simulink model "YMBOX_Deluxe_sim"  (R2024b)
settings: Solver=FixedStepDiscrete  StartTime=0.0  StopTime=YMBOX_Drive_Config.Execution.StopTime_s  FixedStep=KfSIM_PowerStageStep_s  RelTol=1e-3
PreLoadFcn:
  | run(fullfile(fileparts(get_param(bdroot,'FileName')), 'YMBOX_Deluxe_init.m'));
InitFcn:
  | YMBOX_InitializeModel('simulation',bdroot);
model workspace (MAT data in the model file):
  KfMDSP_DCBusVoltFilterCutoff_Hz = Simulink.Parameter
  KfMDSP_DCBusVoltFilterCutoff_Hz.Value = 500
  KfMDSP_DCBusVoltFilterCutoff_Hz.Complexity = 'real'
  KfMDSP_DCBusVoltFilterCutoff_Hz.Dimensions = [1 1]
  KfMDSP_DCBusVoltFilterCutoff_Hz.Description = 'DC bus voltage low-pass cutoff frequency in Hz'
  KfMDSP_DCBusVoltFilterCutoff_Hz.DataType = 'single'
  KfMDSP_DCBusVoltFilterCutoff_Hz.Min = 10
  KfMDSP_DCBusVoltFilterCutoff_Hz.Max = 1000
undefined symbols (not defined in the file or in its folder): Cf_CONTROL_TASK_TIME_S, Cf_TICK_TIME_S, KfPLL_PositionCountsPerRev_NULL, KfSIM_PowerStageStep_s, KfSIM_PwmPeriod_s, KuSIM_PwmDeadTimeSteps_NULL, YMBOX_Drive_Config
libraries: simulink x3, spsDCVoltageSourceLib x1, spsPermanentMagnetSynchronousMachineLib x1, spsUniversalBridgeLib x1, spspowerguiLib x1
CloseFcn:
  | YMBOX_Deluxe_exit
settings Model: Creator=ASUS  LastModifiedBy=ASUS
settings SolverCC: AlgebraicLoopSolver=TrustRegion  AutoInsertRateTranBlk=on
settings DataIOCC: LimitDataPoints=on  SaveFormat=StructureWithTime  SignalLoggingSaveFormat=ModelDataLogs  SaveOutput=off  SaveTime=off  ReturnWorkspaceOutputs=off
settings OptimizationCC: BlockReduction=off  ConditionallyExecuteInputs=off  DefaultParameterBehavior=Inlined  EnhancedBackFolding=on  PassReuseOutputArgsAs=Individual arguments  ExpressionDepthLimit=2147483647  ZeroExternalMemoryAtStartup=off  ZeroInternalMemoryAtStartup=off  InitFltsAndDblsToZero=on  EfficientFloat2IntCast=on  EfficientMapNaN2IntZero=off  OptimizeBlockOrder=speed  DifferentSizesBufferReuse=on  OptimizationCustomize=off  EfficientTunableParamExpr=on
settings DebuggingCC: ConsistencyChecking=warning  ArrayBoundsChecking=error  SignalInfNanChecking=error  SignalRangeChecking=error  SaveWithParameterizedLinksMsg=none  CheckSSInitialOutputMsg=off  UnderspecifiedInitializationDetection=Classic  MergeDetectMultiDrivingBlocksExec=none  TimeAdjustmentMsg=warning  MaxConsecutiveZCsMsg=warning  SolverPrmCheckMsg=warning  InheritedTsInSrcMsg=none  CheckMatrixSingularityMsg=error  ParameterOverflowMsg=warning  ParameterUnderflowMsg=error  ParameterPrecisionLossMsg=none  ParameterTunabilityLossMsg=error  FixptConstUnderflowMsg=warning  FixptConstOverflowMsg=warning  FixptConstPrecisionLossMsg=warning  VectorMatrixConversionMsg=warning  FcnCallInpInsideContextMsg=warning  UnconnectedInputMsg=warning  UnconnectedOutputMsg=warning  UnconnectedLineMsg=warning  UniqueDataStoreMsg=warning  AllowSymbolicDim=off  StateNameClashWarn=warning  SFUnexpectedBacktrackingDiag=warning  SFNoUnconditionalDefaultTransitionDiag=warning  SFExecutionAtInitializationDiag=none  ArithmeticOperatorsInVariantConditions=warning
settings HardwareCC: ProdBitPerPointer=32  ProdBitPerSizeT=32  ProdBitPerPtrDiffT=32  ProdLargestAtomicFloat=None  ProdWordSize=32  ProdHWDeviceType=Infineon->TriCore  TargetIntDivRoundTo=Zero  TargetEndianess=LittleEndian  TargetHWDeviceType=Infineon->TriCore  ProdEqTarget=off
settings ModelReferenceCC: EnableRefExpFcnMdlSchedulingChecks=on  PropagateSignalLabelsOutOfModel=off
settings SFSimCC: SimUseLocalCustomCode=off  MATLABDynamicMemAlloc=off  CustomCodeUndefinedFunction=UseInterfaceOnly
settings SFSimCC: SimCustomSourceCode=|
  | void Pwm_SetOutputToIdle_Now(void){};
  | void InverterDisable(void){};
  | void Pwm_Write(void){};
  | void InverterEnable(void){};
  | void vPwm_MDCC_UdUqCalc1_PI_Self_initialize(void){};
  | void SpeedLoopMode_initialize(void){};
settings SFSimCC: SimCustomHeaderCode=|
  | void Pwm_SetOutputToIdle_Now(void);
  | void InverterDisable(void);
  | void Pwm_Write(void);
  | void InverterEnable(void);
  | void vPwm_MDCC_UdUqCalc1_PI_Self_initialize(void);
  | void SpeedLoopMode_initialize(void);
settings RTWCC: Description=Embedded Coder  SystemTargetFile=ert.tlc  TLCOptions=-p0  GenCodeOnly=on  TemplateMakefile=ert_default_tmf  GenerateReport=on  RTWUseLocalCustomCode=off  IncludeHyperlinkInReport=on  LaunchReport=on  GPUComputeCapability=3.5
settings RTWCC: CustomHeaderCode=|
  | extern void Pwm_SetOutputToIdle_Now(void);
  | extern void InverterDisable(void);
  | extern void Pwm_Write(void);
  | extern void InverterEnable(void);
  | void vPwm_MDCC_UdUqCalc1_PI_Self_initialize(void);
  | void SpeedLoopMode_initialize(void);
settings CodeAppCC: ForceParamTrailComments=on  IgnoreCustomStorageClasses=off  MaxIdLength=100  OperatorAnnotations=on  SimulinkDataObjDesc=on  SFDataObjDesc=on  CustomSymbolStrGlobalVar=rt$N$M  CustomSymbolStrType=$N$M  CustomSymbolStrFcn=$N$M$F  CustomSymbolStrMacro=$N$M  CustomCommentsFcn=comments_mptfun.m  DefineNamingRule=UpperCase  InsertBlockDesc=on  InternalIdentifier=Classic
settings ERTTargetCC: GenerateSampleERTMain=on  ERTCustomFileTemplate=example_file_process.tlc
settings ConfigComp: CovMetricSettings=dw  CovSaveCumulativeToWorkspaceVar=on  CovSaveSingleToWorkspaceVar=on  CovExternalEMLEnable=off

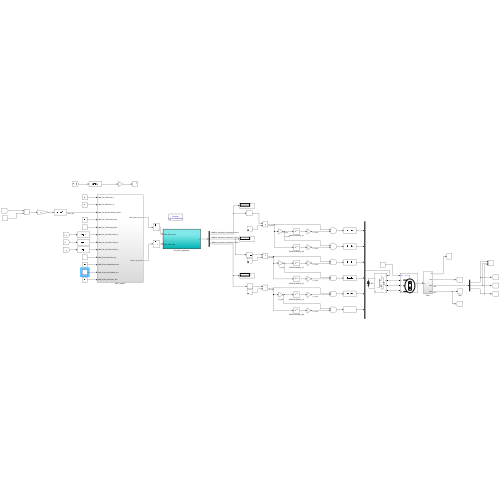
[thumbnail: Simulink's stored preview of the top-level diagram]
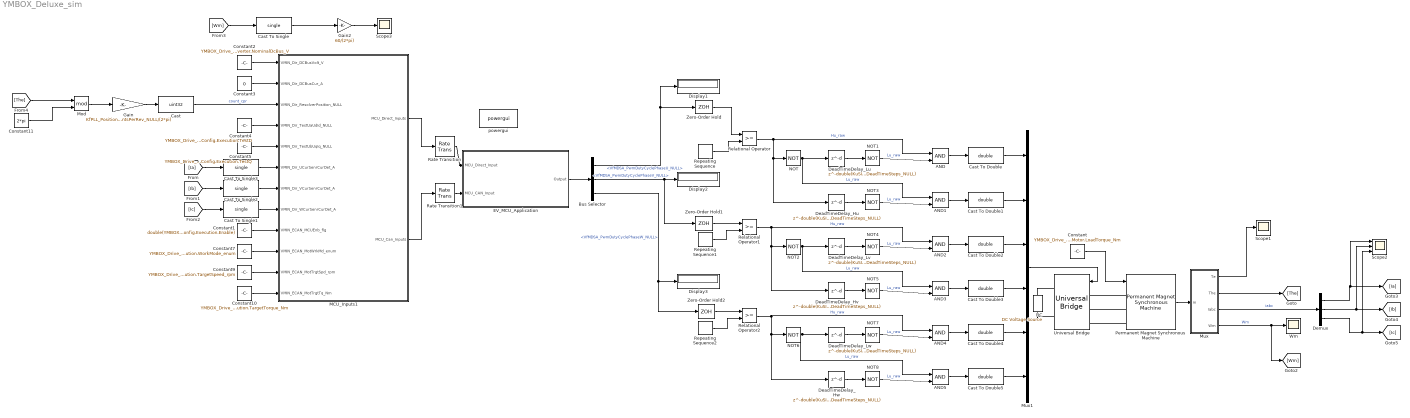
== system YMBOX_Deluxe_sim ==
  AND{,1..5} (6 alike) : Logic  IconShape=distinctive  AllPortsSameDT=off  OutDataTypeStr=boolean
  Bus Selector : BusSelector  OutputSignals=MDSA_output.VfMDSA_PwmDutyCyclePhaseU_NULL,MDSA_output.VfMDSA_PwmDutyCyclePhaseV_NULL,MDSA_output.VfMDSA_PwmDutyCyclePhaseW_NULL
  Cast : DataTypeConversion  OutDataTypeStr=uint32  SaturateOnIntegerOverflow=off  RndMeth=Floor
  Cast To Double{,1..5} (6 alike) : DataTypeConversion  OutDataTypeStr=double  SaturateOnIntegerOverflow=off  RndMeth=Floor
  Cast To Single{,1..3} (4 alike) : DataTypeConversion  OutDataTypeStr=single  SaturateOnIntegerOverflow=off  RndMeth=Floor
  Constant : Constant  Value=YMBOX_Drive_Config.Motor.LoadTorque_Nm
  Constant1 : Constant  Value=double(YMBOX_Drive_Config.Execution.Enable)  OutDataTypeStr=boolean
  Constant10 : Constant  Value=YMBOX_Drive_Config.Execution.TargetTorque_Nm  OutDataTypeStr=single
  Constant11 : Constant  Value=2*pi
  Constant2 : Constant  Value=YMBOX_Drive_Config.Inverter.NominalDcBus_V  OutDataTypeStr=single
  Constant3 : Constant  Value=0  OutDataTypeStr=single
  Constant4 : Constant  Value=YMBOX_Drive_Config.Execution.TestD  OutDataTypeStr=single
  Constant5 : Constant  Value=YMBOX_Drive_Config.Execution.TestQ  OutDataTypeStr=single
  Constant7 : Constant  Value=YMBOX_Drive_Config.Execution.WorkMode_enum  OutDataTypeStr=uint16
  Constant9 : Constant  Value=YMBOX_Drive_Config.Execution.TargetSpeed_rpm  OutDataTypeStr=single
  DC : spsDCVoltageSourceLib/DC Voltage Source  Amplitude=YMBOX_Drive_Config.Inverter.NominalDcBus_V  Measurements=None
  DeadTimeDelay_Hu : Delay  DelayLength=double(KuSIM_PwmDeadTimeSteps_NULL)  InitialCondition=0  SampleTime=KfSIM_PowerStageStep_s
  DeadTimeDelay_Hv : Delay  DelayLength=double(KuSIM_PwmDeadTimeSteps_NULL)  InitialCondition=0  SampleTime=KfSIM_PowerStageStep_s
  DeadTimeDelay_Hw : Delay  DelayLength=double(KuSIM_PwmDeadTimeSteps_NULL)  InitialCondition=0  SampleTime=KfSIM_PowerStageStep_s
  DeadTimeDelay_Lu : Delay  DelayLength=double(KuSIM_PwmDeadTimeSteps_NULL)  InitialCondition=0  SampleTime=KfSIM_PowerStageStep_s
  DeadTimeDelay_Lv : Delay  DelayLength=double(KuSIM_PwmDeadTimeSteps_NULL)  InitialCondition=0  SampleTime=KfSIM_PowerStageStep_s
  DeadTimeDelay_Lw : Delay  DelayLength=double(KuSIM_PwmDeadTimeSteps_NULL)  InitialCondition=0  SampleTime=KfSIM_PowerStageStep_s
  Demux : Demux  Outputs=3
  Display1 : Display
  Display2 : Display
  Display3 : Display
  EV_MCU_Application : Subsystem  TreatAsAtomicUnit=on
      settings: RTWSystemCode=Nonreusable function  RTWFcnNameOpts=Use subsystem name  RTWFileNameOpts=Use subsystem name
  Gain : Gain  Gain=KfPLL_PositionCountsPerRev_NULL/(2*pi)
  Gain2 : Gain  Gain=60/(2*pi)
  MCU_Inputs1 : Subsystem
      settings: RTWSystemCode=Nonreusable function  RTWFcnNameOpts=Use subsystem name  RTWFileNameOpts=Use subsystem name
  Mod : Math  Operator=mod
  Mux : Subsystem
  Mux1 : Mux  Inputs=6
  NOT{,1..8} (9 alike) : Logic  Operator=NOT  IconShape=distinctive  AllPortsSameDT=off  OutDataTypeStr=boolean
  Permanent Magnet Synchronous Machine : spsPermanentMagnetSynchronousMachineLib/Permanent Magnet Synchronous Machine  NbPhases=3  FluxDistribution=Sinusoidal  RotorType=Salient-pole  MechanicalLoad=Torque Tm  PresetModel=No  ShowDetailedParameters=on  MeasurementBus=off  Resistance=YMBOX_Drive_Config.Motor.StatorResistance_Ohm  Inductance=8.5e-3  dqInductances=[YMBOX_Drive_Config.Motor.Ld_H YMBOX_Drive_Config.Motor.Lq_H]  La=YMBOX_Drive_Config.Motor.Ld_H  MachineConstant=Flux linkage established by magnets (V.s)  Flux=YMBOX_Drive_Config.Motor.PmFlux_Wb  VoltageCst=68.3065  TorqueCst=0.56489  Flat=120  Mechanical=[YMBOX_Drive_Config.Motor.Inertia_kgm2 YMBOX_Drive_Config.Motor.ViscousFriction_Nms YMBOX_Drive_Config.Motor.PolePairs 0]  PolePairs=YMBOX_Drive_Config.Motor.PolePairs  InitialConditions=[0,0, 0,0]  InitialConditions5ph=[0 0 0 0 0 0]  RefAngle=Aligned with phase A axis (original Park)  IterativeDiscreteModel=Trapezoidal non iterative  TsBlock=-1  TsPowergui=0
  Rate Transition : RateTransition  OutPortSampleTime=Cf_CONTROL_TASK_TIME_S
  Rate Transition1 : RateTransition  OutPortSampleTime=Cf_CONTROL_TASK_TIME_S
  Relational Operator : RelationalOperator  OutDataTypeStr=boolean  RndMeth=Simplest  InputSameDT=off
  Relational Operator1 : RelationalOperator  OutDataTypeStr=boolean  RndMeth=Simplest  InputSameDT=off
  Relational Operator2 : RelationalOperator  OutDataTypeStr=boolean  RndMeth=Simplest  InputSameDT=off
  Repeating Sequence : simulink/Sources/Repeating Sequence  rep_seq_t=[0 0.5*KfSIM_PwmPeriod_s KfSIM_PwmPeriod_s]  rep_seq_y=[0 1 0]
  Repeating Sequence1 : simulink/Sources/Repeating Sequence  rep_seq_t=[0 0.5*KfSIM_PwmPeriod_s KfSIM_PwmPeriod_s]  rep_seq_y=[0 1 0]
  Repeating Sequence2 : simulink/Sources/Repeating Sequence  rep_seq_t=[0 0.5*KfSIM_PwmPeriod_s KfSIM_PwmPeriod_s]  rep_seq_y=[0 1 0]
  Scope1 : Scope
  Scope2 : Scope  NumInputPorts=3
  Scope3 : Scope
  Universal Bridge : spsUniversalBridgeLib/Universal Bridge  Arms=3  SnubberResistance=1e5  SnubberCapacitance=inf  Device=IGBT / Diodes  Ron=1e-3  Lon=0  ForwardVoltages="[  0  0  ]"  ForwardVoltage=0  GTOparameters=[ 10e-6 , 20e-6 ]  IGBTparameters=[ 1e-6 , 2e-6 ]  Measurements=None  Measurements_2=None  converterType=Rectifier
  Wm : Scope
  Zero-Order Hold : ZeroOrderHold  SampleTime=Cf_CONTROL_TASK_TIME_S
  Zero-Order Hold1 : ZeroOrderHold  SampleTime=Cf_CONTROL_TASK_TIME_S
  Zero-Order Hold2 : ZeroOrderHold  SampleTime=Cf_CONTROL_TASK_TIME_S
  powergui : spspowerguiLib/powergui  Priority=1  SimulationMode=Discrete  SampleTime=KfSIM_PowerStageStep_s  frequency=60  Iterations=50  frequencyindice=0  Pbase=100e6  ErrMax=1e-4  UnitsV=kV  UnitsW=MW  buscounter=0  FunctionMessages=off  echomessages=off  EnableUseOfTLC=off  CurrentSourceSwitches=off  DisableSnubberDevices=off  DisableRonSwitches=off  DisableVfSwitches=off  DisplayEquations=off  AutomaticDiscreteSolvers=off  SolverType=Tustin/Backward Euler (TBE)  Interpol=off  ExternalGateDelay=off  methode=off  Ts=100  x0status=blocks  SPID=on  SwTol=0  HookPort=off  NonlinearTolerance=1e-4  nMaxIteration=100  ContinueOnMaxIteration=off  RestoreLinks=warning  ResistiveCurrentMeasurement=off  Frange=[0:2:500]  Ylog=off  Xlog=on  ShowGrid=off  save=off  variable=ZData  structure=0  ZoomFFT=off  StartTime=0.0  cycles=1  DisplayStyle=1  fundamental=60  FreqAxis=off  MaxFrequency=1000  frequencyindicesteady=1  RmsSteady=1  display=off
  wires:
  NOT6/1 -> AND5/1, DeadTimeDelay_Lw/1  "Lu_raw"
  Bus Selector/1 -> Display1/1, Zero-Order Hold/1  "<VfMDSA_PwmDutyCyclePhaseU_NULL>"
  Mux/4(Wm) -> [Wm], Wm/1  "Wm"
  [Ic] -> Cast To Single1/1
  Zero-Order Hold/1 -> Relational Operator/1
  Repeating Sequence2/1 -> Relational Operator2/2
  AND1/1 -> Cast To Double1/1
  AND/1 -> Cast To Double/1
  Mux/2(The) -> [The]
  [The] -> Mod/1
  Cast To Single/1 -> Gain2/1
  AND2/1 -> Cast To Double2/1
  Relational Operator1/1 -> AND2/1, DeadTimeDelay_Hv/1, NOT2/1  "Hu_raw"
  Demux/1 -> Scope2/1, [Ia]
  Relational Operator2/1 -> AND4/1, DeadTimeDelay_Hw/1, NOT6/1  "Hu_raw"
  Bus Selector/2 -> Zero-Order Hold1/1, Display2/1  "<VfMDSA_PwmDutyCyclePhaseV_NULL>"
  NOT8/1 -> AND5/2  "Lu_raw"
  NOT7/1 -> AND4/2  "Lu_raw"
  Cast To Double2/1 -> Mux1/3
  Cast To Single1/1 -> MCU_Inputs1/8(VMIN_Dir_WCurSenrCurDet_A)
  Constant3/1 -> MCU_Inputs1/2(VMIN_Dir_DCBusCur_A)
  Constant1/1 -> MCU_Inputs1/9(VMIN_ECAN_MCUEnb_flg)
  Zero-Order Hold1/1 -> Relational Operator1/1
  Constant/1 -> Permanent Magnet Synchronous Machine/1
  [Ib] -> Cast To Single2/1
  Constant5/1 -> MCU_Inputs1/5(VMIN_Dir_TestUbUqIq_NULL)
  NOT2/1 -> AND3/1, DeadTimeDelay_Lv/1  "Lu_raw"
  Gain2/1 -> Scope3/1
  Cast To Double/1 -> Mux1/1
  Constant10/1 -> MCU_Inputs1/12(VMIN_ECAN_MotTrgtTq_Nm)
  Cast To Single2/1 -> MCU_Inputs1/7(VMIN_Dir_VCurSenrCurDet_A)
  Permanent Magnet Synchronous Machine/1 -> Mux/1(m)
  Constant7/1 -> MCU_Inputs1/10(VMIN_ECAN_MotWrkMd_enum)
  Cast To Double1/1 -> Mux1/2
  Zero-Order Hold2/1 -> Relational Operator2/1
  Constant4/1 -> MCU_Inputs1/4(VMIN_Dir_TestUaUdId_NULL)
  Mux/1(Te) -> Scope1/1
  Demux/3 -> Scope2/3, [Ic]
  Constant2/1 -> MCU_Inputs1/1(VMIN_Dir_DCBusVolt_V)
  AND4/1 -> Cast To Double4/1
  Mod/1 -> Gain/1
  Cast To Double3/1 -> Mux1/4
  EV_MCU_Application/1(Output) -> Bus Selector/1
  NOT3/1 -> AND1/2  "Lu_raw"
  Demux/2 -> Scope2/2, [Ib]
  Cast To Single3/1 -> MCU_Inputs1/6(VMIN_Dir_UCurSenrCurDet_A)
  AND5/1 -> Cast To Double5/1
  NOT1/1 -> AND/2  "Lu_raw"
  Mux/3(Iabc) -> Demux/1  "iabc"
  Cast/1 -> MCU_Inputs1/3(VMIN_Dir_ResolverPosition_NULL)  "count_cpr"
  Gain/1 -> Cast/1
  Cast To Double5/1 -> Mux1/6
  NOT/1 -> AND1/1, DeadTimeDelay_Lu/1  "Lu_raw"
  Constant9/1 -> MCU_Inputs1/11(VMIN_ECAN_MotTrgtSpd_rpm)
  Mux1/1 -> Universal Bridge/1
  Constant11/1 -> Mod/2
  NOT4/1 -> AND2/2  "Lu_raw"
  Cast To Double4/1 -> Mux1/5
  NOT5/1 -> AND3/2  "Lu_raw"
  [Wm] -> Cast To Single/1
  Relational Operator/1 -> AND/1, DeadTimeDelay_Hu/1, NOT/1  "Hu_raw"
  Bus Selector/3 -> Zero-Order Hold2/1, Display3/1  "<VfMDSA_PwmDutyCyclePhaseW_NULL>"
  Repeating Sequence/1 -> Relational Operator/2
  AND3/1 -> Cast To Double3/1
  [Ia] -> Cast To Single3/1
  Repeating Sequence1/1 -> Relational Operator1/2
  MCU_Inputs1/1(MCU_Direct_Inputs) -> Rate Transition/1
  Rate Transition/1 -> EV_MCU_Application/1(MCU_Direct_Input)
  Rate Transition1/1 -> EV_MCU_Application/2(MCU_CAN_Input)
  MCU_Inputs1/2(MCU_Can_Inputs) -> Rate Transition1/1
  DeadTimeDelay_Lu/1 -> NOT1/1
  DeadTimeDelay_Hu/1 -> NOT3/1
  DeadTimeDelay_Lv/1 -> NOT4/1
  DeadTimeDelay_Hv/1 -> NOT5/1
  DeadTimeDelay_Lw/1 -> NOT7/1
  DeadTimeDelay_Hw/1 -> NOT8/1
  connections:
  DC/LConn1 -- Universal Bridge/RConn2
  DC/RConn1 -- Universal Bridge/RConn1
  Permanent Magnet Synchronous Machine/LConn3 -- Universal Bridge/LConn3
  Permanent Magnet Synchronous Machine/LConn1 -- Universal Bridge/LConn1
  Permanent Magnet Synchronous Machine/LConn2 -- Universal Bridge/LConn2

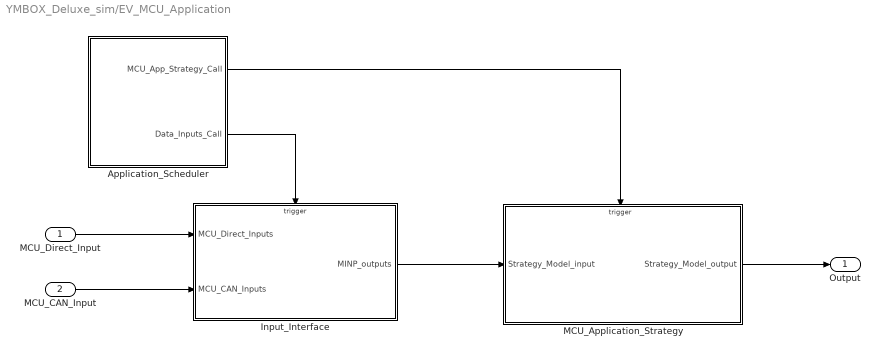
== system YMBOX_Deluxe_sim/EV_MCU_Application ==
  MCU_Direct_Input : Inport
  MCU_CAN_Input : Inport  Port=2
  Application_Scheduler : Subsystem
  Input_Interface : Subsystem
      settings: RTWSystemCode=Nonreusable function  RTWFcnNameOpts=Use subsystem name  RTWFileNameOpts=Use subsystem name
  MCU_Application_Strategy : Subsystem
      settings: RTWSystemCode=Nonreusable function  RTWFcnNameOpts=Use subsystem name  RTWFileNameOpts=Use subsystem name
  Output : Outport
  wires:
  MCU_Direct_Input/1 -> Input_Interface/1(MCU_Direct_Inputs)
  MCU_CAN_Input/1 -> Input_Interface/2(MCU_CAN_Inputs)
  Input_Interface/1(MINP_outputs) -> MCU_Application_Strategy/1(Strategy_Model_input)
  MCU_Application_Strategy/1(Strategy_Model_output) -> Output/1
  Application_Scheduler/1(MCU_App_Strategy_Call) -> MCU_Application_Strategy/Trigger
  Application_Scheduler/2(Data_Inputs_Call) -> Input_Interface/Trigger

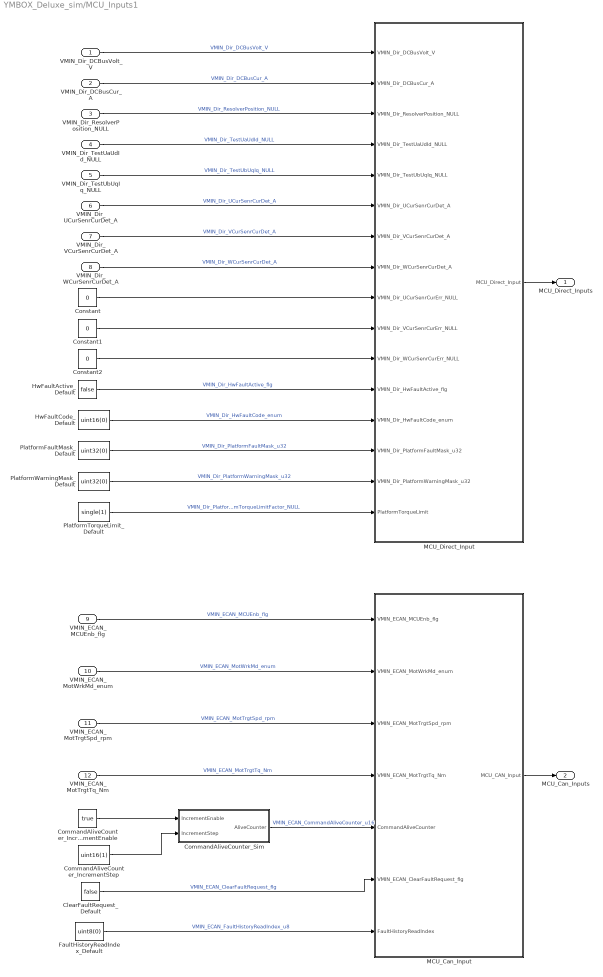
== system YMBOX_Deluxe_sim/MCU_Inputs1 ==
  VMIN_Dir_DCBusVolt_V : Inport
  VMIN_Dir_DCBusCur_A : Inport  Port=2
  VMIN_Dir_ResolverPosition_NULL : Inport  Port=3
  VMIN_Dir_TestUaUdId_NULL : Inport  Port=4
  VMIN_Dir_TestUbUqIq_NULL : Inport  Port=5
  VMIN_Dir_UCurSenrCurDet_A : Inport  Port=6
  VMIN_Dir_VCurSenrCurDet_A : Inport  Port=7
  VMIN_Dir_WCurSenrCurDet_A : Inport  Port=8
  VMIN_ECAN_MCUEnb_flg : Inport  Port=9
  VMIN_ECAN_MotWrkMd_enum : Inport  Port=10
  VMIN_ECAN_MotTrgtSpd_rpm : Inport  Port=11
  VMIN_ECAN_MotTrgtTq_Nm : Inport  Port=12
  ClearFaultRequest_Default : Constant  Value=false  OutDataTypeStr=boolean
  CommandAliveCounter_IncrementEnable : Constant  Description=仿真控制：true 时 AliveCounter 按步长递增；false 时保持当前值，用于触发 CommWatchdog 停更场景。  Value=true  OutDataTypeStr=boolean
  CommandAliveCounter_IncrementStep : Constant  Description=仿真控制：AliveCounter 每个控制节拍的 uint16 增量，默认 uint16(1)。  Value=uint16(1)  OutDataTypeStr=uint16
  CommandAliveCounter_Sim : Subsystem  Description=仿真专用命令存活计数器：Enable 有效时每个 Cf_TICK_TIME_S 加 IncrementStep；无效时保持；uint16 溢出自然回绕。
  Constant : Constant  Value=0  OutDataTypeStr=boolean
  Constant1 : Constant  Value=0  OutDataTypeStr=boolean
  Constant2 : Constant  Value=0  OutDataTypeStr=boolean
  FaultHistoryReadIndex_Default : Constant  Value=uint8(0)  OutDataTypeStr=uint8
  HwFaultActive_Default : Constant  Value=false  OutDataTypeStr=boolean
  HwFaultCode_Default : Constant  Value=uint16(0)  OutDataTypeStr=uint16
  MCU_Can_Input : Subsystem  TreatAsAtomicUnit=on
      settings: RTWSystemCode=Nonreusable function  RTWFcnNameOpts=Use subsystem name
  MCU_Direct_Input : Subsystem  TreatAsAtomicUnit=on
      settings: RTWSystemCode=Nonreusable function  RTWFcnNameOpts=Use subsystem name
  PlatformFaultMask_Default : Constant  Value=uint32(0)  OutDataTypeStr=uint32
  PlatformTorqueLimit_Default : Constant  Value=single(1)  OutDataTypeStr=single
  PlatformWarningMask_Default : Constant  Value=uint32(0)  OutDataTypeStr=uint32
  MCU_Direct_Inputs : Outport
  MCU_Can_Inputs : Outport  Port=2
  wires:
  VMIN_Dir_DCBusVolt_V/1 -> MCU_Direct_Input/1(VMIN_Dir_DCBusVolt_V)  "VMIN_Dir_DCBusVolt_V"
  VMIN_Dir_TestUbUqIq_NULL/1 -> MCU_Direct_Input/5(VMIN_Dir_TestUbUqIq_NULL)  "VMIN_Dir_TestUbUqIq_NULL"
  VMIN_Dir_TestUaUdId_NULL/1 -> MCU_Direct_Input/4(VMIN_Dir_TestUaUdId_NULL)  "VMIN_Dir_TestUaUdId_NULL"
  VMIN_Dir_ResolverPosition_NULL/1 -> MCU_Direct_Input/3(VMIN_Dir_ResolverPosition_NULL)  "VMIN_Dir_ResolverPosition_NULL"
  VMIN_Dir_DCBusCur_A/1 -> MCU_Direct_Input/2(VMIN_Dir_DCBusCur_A)  "VMIN_Dir_DCBusCur_A"
  VMIN_ECAN_MotTrgtTq_Nm/1 -> MCU_Can_Input/4(VMIN_ECAN_MotTrgtTq_Nm)  "VMIN_ECAN_MotTrgtTq_Nm"
  HwFaultCode_Default/1 -> MCU_Direct_Input/13(VMIN_Dir_HwFaultCode_enum)  "VMIN_Dir_HwFaultCode_enum"
  Constant1/1 -> MCU_Direct_Input/10(VMIN_Dir_VCurSenrCurErr_NULL)
  VMIN_Dir_WCurSenrCurDet_A/1 -> MCU_Direct_Input/8(VMIN_Dir_WCurSenrCurDet_A)  "VMIN_Dir_WCurSenrCurDet_A"
  HwFaultActive_Default/1 -> MCU_Direct_Input/12(VMIN_Dir_HwFaultActive_flg)  "VMIN_Dir_HwFaultActive_flg"
  Constant/1 -> MCU_Direct_Input/9(VMIN_Dir_UCurSenrCurErr_NULL)
  VMIN_Dir_VCurSenrCurDet_A/1 -> MCU_Direct_Input/7(VMIN_Dir_VCurSenrCurDet_A)  "VMIN_Dir_VCurSenrCurDet_A"
  VMIN_Dir_UCurSenrCurDet_A/1 -> MCU_Direct_Input/6(VMIN_Dir_UCurSenrCurDet_A)  "VMIN_Dir_UCurSenrCurDet_A"
  MCU_Can_Input/1(MCU_CAN_Input) -> MCU_Can_Inputs/1
  VMIN_ECAN_MCUEnb_flg/1 -> MCU_Can_Input/1(VMIN_ECAN_MCUEnb_flg)  "VMIN_ECAN_MCUEnb_flg"
  Constant2/1 -> MCU_Direct_Input/11(VMIN_Dir_WCurSenrCurErr_NULL)
  PlatformFaultMask_Default/1 -> MCU_Direct_Input/14(VMIN_Dir_PlatformFaultMask_u32)  "VMIN_Dir_PlatformFaultMask_u32"
  PlatformWarningMask_Default/1 -> MCU_Direct_Input/15(VMIN_Dir_PlatformWarningMask_u32)  "VMIN_Dir_PlatformWarningMask_u32"
  PlatformTorqueLimit_Default/1 -> MCU_Direct_Input/16(PlatformTorqueLimit)  "VMIN_Dir_PlatformTorqueLimitFactor_NULL"
  FaultHistoryReadIndex_Default/1 -> MCU_Can_Input/7(FaultHistoryReadIndex)  "VMIN_ECAN_FaultHistoryReadIndex_u8"
  VMIN_ECAN_MotWrkMd_enum/1 -> MCU_Can_Input/2(VMIN_ECAN_MotWrkMd_enum)  "VMIN_ECAN_MotWrkMd_enum"
  VMIN_ECAN_MotTrgtSpd_rpm/1 -> MCU_Can_Input/3(VMIN_ECAN_MotTrgtSpd_rpm)  "VMIN_ECAN_MotTrgtSpd_rpm"
  ClearFaultRequest_Default/1 -> MCU_Can_Input/6(VMIN_ECAN_ClearFaultRequest_flg)  "VMIN_ECAN_ClearFaultRequest_flg"
  MCU_Direct_Input/1(MCU_Direct_Input) -> MCU_Direct_Inputs/1
  CommandAliveCounter_IncrementEnable/1 -> CommandAliveCounter_Sim/1(IncrementEnable)
  CommandAliveCounter_IncrementStep/1 -> CommandAliveCounter_Sim/2(IncrementStep)
  CommandAliveCounter_Sim/1(AliveCounter) -> MCU_Can_Input/5(CommandAliveCounter)  "VMIN_ECAN_CommandAliveCounter_u16"

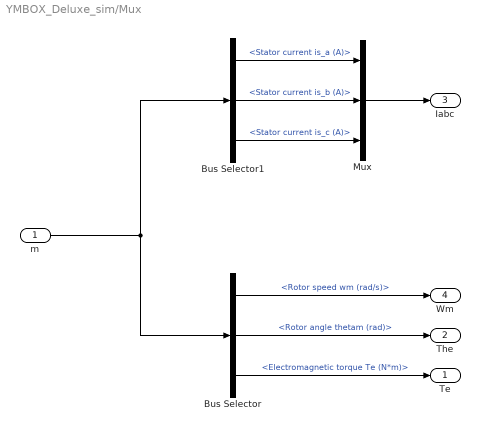
== system YMBOX_Deluxe_sim/Mux ==
  m : Inport
  Bus Selector : BusSelector  OutputSignals=Rotor speed wm (rad/s),Rotor angle thetam (rad),Electromagnetic torque Te (N*m)
  Bus Selector1 : BusSelector  OutputSignals=Stator current is_a (A),Stator current is_b (A),Stator current is_c (A)
  Mux : Mux  Inputs=3
  Te : Outport
  The : Outport  Port=2
  Iabc : Outport  Port=3
  Wm : Outport  Port=4
  wires:
  m/1 -> Bus Selector/1, Bus Selector1/1
  Bus Selector/2 -> The/1  "<Rotor angle thetam (rad)>"
  Bus Selector/3 -> Te/1  "<Electromagnetic torque Te (N*m)>"
  Bus Selector/1 -> Wm/1  "<Rotor speed wm (rad/s)>"
  Bus Selector1/1 -> Mux/1  "<Stator current is_a (A)>"
  Bus Selector1/2 -> Mux/2  "<Stator current is_b (A)>"
  Bus Selector1/3 -> Mux/3  "<Stator current is_c (A)>"
  Mux/1 -> Iabc/1

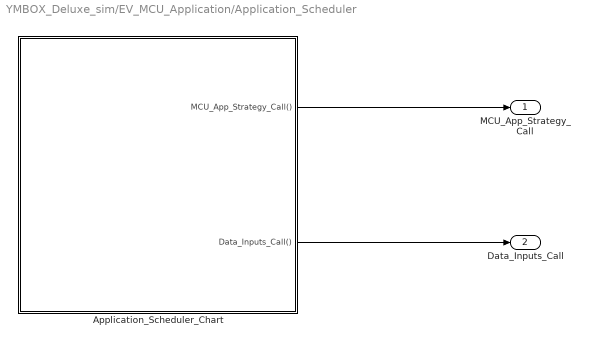
== system YMBOX_Deluxe_sim/EV_MCU_Application/Application_Scheduler ==
  Application_Scheduler_Chart : Stateflow chart  TreatAsAtomicUnit=on
      settings: CopyFcn=set_param(gcb,'linkstatus','None');
  MCU_App_Strategy_Call : Outport
  Data_Inputs_Call : Outport  Port=2
  wires:
  Application_Scheduler_Chart/1(MCU_App_Strategy_Call()) -> MCU_App_Strategy_Call/1
  Application_Scheduler_Chart/2(Data_Inputs_Call()) -> Data_Inputs_Call/1

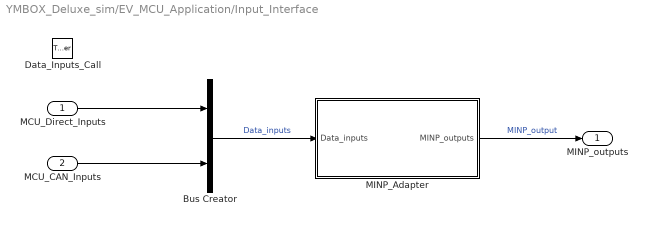
== system YMBOX_Deluxe_sim/EV_MCU_Application/Input_Interface ==
  MCU_Direct_Inputs : Inport
  MCU_CAN_Inputs : Inport  Port=2
  Data_Inputs_Call : TriggerPort  TriggerType=function-call  VariantControl=(inherit)
  Bus Creator : BusCreator  Inputs=2
  MINP_Adapter : Subsystem
      settings: RTWSystemCode=Nonreusable function  RTWFcnNameOpts=Use subsystem name
  MINP_outputs : Outport  OutDataTypeStr=Bus: MINP_output
  wires:
  Bus Creator/1 -> MINP_Adapter/1(Data_inputs)  "Data_inputs"
  MCU_CAN_Inputs/1 -> Bus Creator/2
  MCU_Direct_Inputs/1 -> Bus Creator/1
  MINP_Adapter/1(MINP_outputs) -> MINP_outputs/1  "MINP_output"

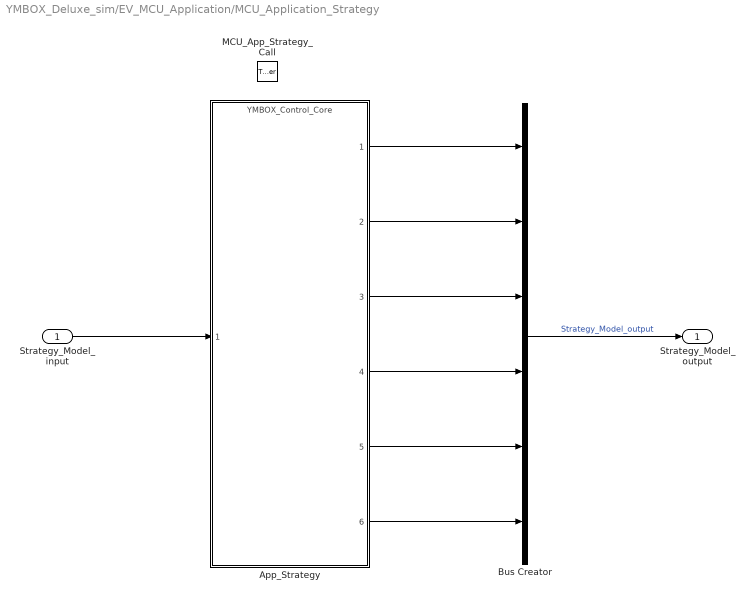
== system YMBOX_Deluxe_sim/EV_MCU_Application/MCU_Application_Strategy ==
  Strategy_Model_input : Inport
  MCU_App_Strategy_Call : TriggerPort  TriggerType=function-call  VariantControl=(inherit)
  App_Strategy : ModelReference  ModelNameDialog=YMBOX_Control_Core  SimulationMode=Normal  ModelReferenceVersion=19.1096
  Bus Creator : BusCreator  Inputs=6
  Strategy_Model_output : Outport
  wires:
  Strategy_Model_input/1 -> App_Strategy/1
  Bus Creator/1 -> Strategy_Model_output/1  "Strategy_Model_output"
  App_Strategy/1 -> Bus Creator/1
  App_Strategy/2 -> Bus Creator/2
  App_Strategy/3 -> Bus Creator/3
  App_Strategy/4 -> Bus Creator/4
  App_Strategy/5 -> Bus Creator/5
  App_Strategy/6 -> Bus Creator/6

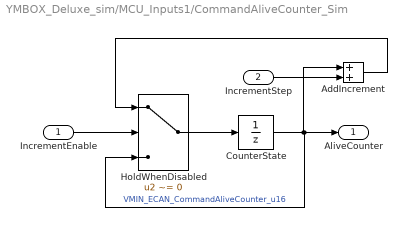
== system YMBOX_Deluxe_sim/MCU_Inputs1/CommandAliveCounter_Sim ==
  IncrementEnable : Inport
  IncrementStep : Inport  Port=2
  AddIncrement : Sum
  CounterState : UnitDelay  InitialCondition=uint16(0)  SampleTime=Cf_TICK_TIME_S
  HoldWhenDisabled : Switch  Criteria=u2 ~= 0
  AliveCounter : Outport
  wires:
  IncrementEnable/1 -> HoldWhenDisabled/2
  HoldWhenDisabled/1 -> CounterState/1
  IncrementStep/1 -> AddIncrement/2
  CounterState/1 -> HoldWhenDisabled/3, AliveCounter/1, AddIncrement/1  "VMIN_ECAN_CommandAliveCounter_u16"
  AddIncrement/1 -> HoldWhenDisabled/1

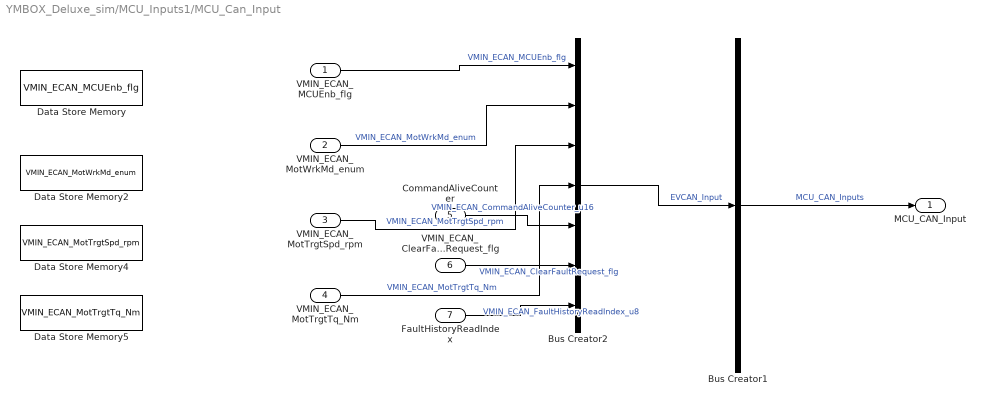
== system YMBOX_Deluxe_sim/MCU_Inputs1/MCU_Can_Input ==
  VMIN_ECAN_MCUEnb_flg : Inport
  VMIN_ECAN_MotWrkMd_enum : Inport  Port=2
  VMIN_ECAN_MotTrgtSpd_rpm : Inport  Port=3
  VMIN_ECAN_MotTrgtTq_Nm : Inport  Port=4
  CommandAliveCounter : Inport  Port=5  OutDataTypeStr=uint16
  VMIN_ECAN_ClearFaultRequest_flg : Inport  Port=6  OutDataTypeStr=boolean
  FaultHistoryReadIndex : Inport  Port=7  OutDataTypeStr=uint8
  Bus Creator1 : BusCreator  Inputs=1
  Bus Creator2 : BusCreator  Inputs=7
  Data Store Memory : DataStoreMemory  DataStoreName=VMIN_ECAN_MCUEnb_flg  WriteAfterWriteMsg=warning  ShowAdditionalParam=off  OutDataTypeStr=boolean
  Data Store Memory2 : DataStoreMemory  DataStoreName=VMIN_ECAN_MotWrkMd_enum  WriteAfterWriteMsg=warning  ShowAdditionalParam=off  OutDataTypeStr=uint16
  Data Store Memory4 : DataStoreMemory  DataStoreName=VMIN_ECAN_MotTrgtSpd_rpm  WriteAfterWriteMsg=warning  ShowAdditionalParam=off  OutDataTypeStr=single
  Data Store Memory5 : DataStoreMemory  DataStoreName=VMIN_ECAN_MotTrgtTq_Nm  WriteAfterWriteMsg=warning  ShowAdditionalParam=off  OutDataTypeStr=single
  MCU_CAN_Input : Outport
  wires:
  Bus Creator2/1 -> Bus Creator1/1  "EVCAN_Input"
  Bus Creator1/1 -> MCU_CAN_Input/1  "MCU_CAN_Inputs"
  VMIN_ECAN_MCUEnb_flg/1 -> Bus Creator2/1  "VMIN_ECAN_MCUEnb_flg"
  VMIN_ECAN_MotWrkMd_enum/1 -> Bus Creator2/2  "VMIN_ECAN_MotWrkMd_enum"
  VMIN_ECAN_MotTrgtSpd_rpm/1 -> Bus Creator2/3  "VMIN_ECAN_MotTrgtSpd_rpm"
  VMIN_ECAN_MotTrgtTq_Nm/1 -> Bus Creator2/4  "VMIN_ECAN_MotTrgtTq_Nm"
  CommandAliveCounter/1 -> Bus Creator2/5  "VMIN_ECAN_CommandAliveCounter_u16"
  VMIN_ECAN_ClearFaultRequest_flg/1 -> Bus Creator2/6  "VMIN_ECAN_ClearFaultRequest_flg"
  FaultHistoryReadIndex/1 -> Bus Creator2/7  "VMIN_ECAN_FaultHistoryReadIndex_u8"

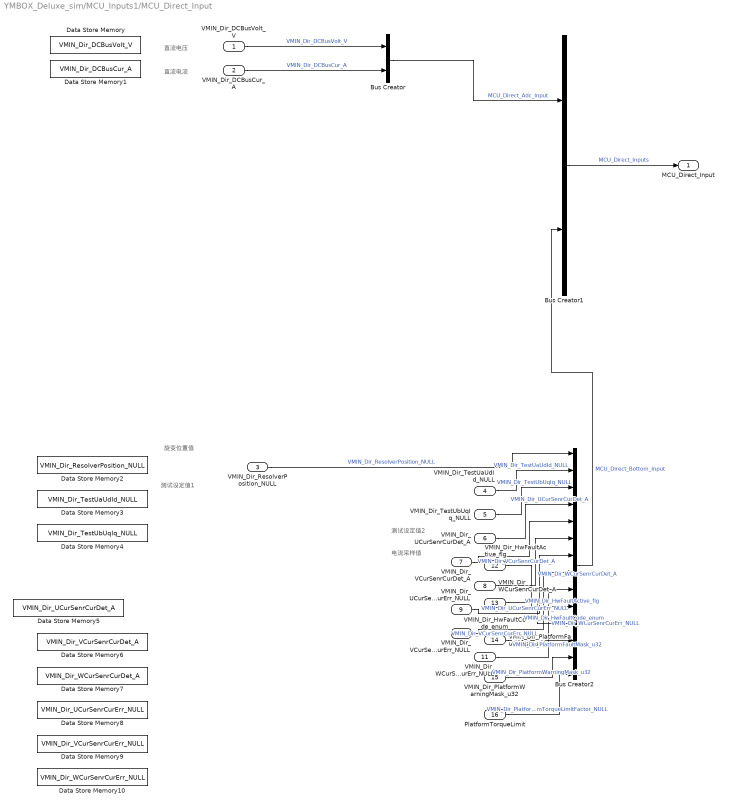
== system YMBOX_Deluxe_sim/MCU_Inputs1/MCU_Direct_Input ==
  note: 直流电压
  note: 直流电流
  note: 旋变位置值
  note: 测试设定值1
  note: 测试设定值2
  note: 电流采样值
  VMIN_Dir_DCBusVolt_V : Inport
  VMIN_Dir_DCBusCur_A : Inport  Port=2
  VMIN_Dir_ResolverPosition_NULL : Inport  Port=3
  VMIN_Dir_TestUaUdId_NULL : Inport  Port=4
  VMIN_Dir_TestUbUqIq_NULL : Inport  Port=5
  VMIN_Dir_UCurSenrCurDet_A : Inport  Port=6
  VMIN_Dir_VCurSenrCurDet_A : Inport  Port=7
  VMIN_Dir_WCurSenrCurDet_A : Inport  Port=8
  VMIN_Dir_UCurSenrCurErr_NULL : Inport  Port=9
  VMIN_Dir_VCurSenrCurErr_NULL : Inport  Port=10
  VMIN_Dir_WCurSenrCurErr_NULL : Inport  Port=11
  VMIN_Dir_HwFaultActive_flg : Inport  Port=12  OutDataTypeStr=boolean
  VMIN_Dir_HwFaultCode_enum : Inport  Port=13  OutDataTypeStr=uint16
  VMIN_Dir_PlatformFaultMask_u32 : Inport  Port=14  OutDataTypeStr=uint32
  VMIN_Dir_PlatformWarningMask_u32 : Inport  Port=15  OutDataTypeStr=uint32
  PlatformTorqueLimit : Inport  Port=16  OutDataTypeStr=single
  Bus Creator : BusCreator  Inputs=2
  Bus Creator1 : BusCreator  Inputs=2
  Bus Creator2 : BusCreator  Inputs=14
  Data Store Memory : DataStoreMemory  DataStoreName=VMIN_Dir_DCBusVolt_V  WriteAfterWriteMsg=warning  ShowAdditionalParam=off  OutDataTypeStr=single
  Data Store Memory1 : DataStoreMemory  DataStoreName=VMIN_Dir_DCBusCur_A  WriteAfterWriteMsg=warning  ShowAdditionalParam=off  OutDataTypeStr=single
  Data Store Memory10 : DataStoreMemory  DataStoreName=VMIN_Dir_WCurSenrCurErr_NULL  WriteAfterWriteMsg=warning  ShowAdditionalParam=off  OutDataTypeStr=boolean
  Data Store Memory2 : DataStoreMemory  DataStoreName=VMIN_Dir_ResolverPosition_NULL  WriteAfterWriteMsg=warning  ShowAdditionalParam=off  OutDataTypeStr=uint16
  Data Store Memory3 : DataStoreMemory  DataStoreName=VMIN_Dir_TestUaUdId_NULL  WriteAfterWriteMsg=warning  ShowAdditionalParam=off  OutDataTypeStr=single
  Data Store Memory4 : DataStoreMemory  DataStoreName=VMIN_Dir_TestUbUqIq_NULL  WriteAfterWriteMsg=warning  ShowAdditionalParam=off  OutDataTypeStr=single
  Data Store Memory5 : DataStoreMemory  DataStoreName=VMIN_Dir_UCurSenrCurDet_A  WriteAfterWriteMsg=warning  ShowAdditionalParam=off  OutDataTypeStr=single
  Data Store Memory6 : DataStoreMemory  DataStoreName=VMIN_Dir_VCurSenrCurDet_A  WriteAfterWriteMsg=warning  ShowAdditionalParam=off  OutDataTypeStr=single
  Data Store Memory7 : DataStoreMemory  DataStoreName=VMIN_Dir_WCurSenrCurDet_A  WriteAfterWriteMsg=warning  ShowAdditionalParam=off  OutDataTypeStr=single
  Data Store Memory8 : DataStoreMemory  DataStoreName=VMIN_Dir_UCurSenrCurErr_NULL  WriteAfterWriteMsg=warning  ShowAdditionalParam=off  OutDataTypeStr=boolean
  Data Store Memory9 : DataStoreMemory  DataStoreName=VMIN_Dir_VCurSenrCurErr_NULL  WriteAfterWriteMsg=warning  ShowAdditionalParam=off  OutDataTypeStr=boolean
  MCU_Direct_Input : Outport
  wires:
  VMIN_Dir_DCBusVolt_V/1 -> Bus Creator/1  "VMIN_Dir_DCBusVolt_V"
  VMIN_Dir_DCBusCur_A/1 -> Bus Creator/2  "VMIN_Dir_DCBusCur_A"
  Bus Creator/1 -> Bus Creator1/1  "MCU_Direct_Adc_Input"
  Bus Creator1/1 -> MCU_Direct_Input/1  "MCU_Direct_Inputs"
  VMIN_Dir_ResolverPosition_NULL/1 -> Bus Creator2/1  "VMIN_Dir_ResolverPosition_NULL"
  VMIN_Dir_TestUaUdId_NULL/1 -> Bus Creator2/2  "VMIN_Dir_TestUaUdId_NULL"
  VMIN_Dir_TestUbUqIq_NULL/1 -> Bus Creator2/3  "VMIN_Dir_TestUbUqIq_NULL"
  Bus Creator2/1 -> Bus Creator1/2  "MCU_Direct_Bottom_Input"
  VMIN_Dir_VCurSenrCurDet_A/1 -> Bus Creator2/5  "VMIN_Dir_VCurSenrCurDet_A"
  VMIN_Dir_UCurSenrCurDet_A/1 -> Bus Creator2/4  "VMIN_Dir_UCurSenrCurDet_A"
  VMIN_Dir_WCurSenrCurDet_A/1 -> Bus Creator2/6  "VMIN_Dir_WCurSenrCurDet_A"
  VMIN_Dir_UCurSenrCurErr_NULL/1 -> Bus Creator2/7  "VMIN_Dir_UCurSenrCurErr_NULL"
  VMIN_Dir_VCurSenrCurErr_NULL/1 -> Bus Creator2/8  "VMIN_Dir_VCurSenrCurErr_NULL"
  VMIN_Dir_WCurSenrCurErr_NULL/1 -> Bus Creator2/9  "VMIN_Dir_WCurSenrCurErr_NULL"
  VMIN_Dir_HwFaultActive_flg/1 -> Bus Creator2/10  "VMIN_Dir_HwFaultActive_flg"
  VMIN_Dir_HwFaultCode_enum/1 -> Bus Creator2/11  "VMIN_Dir_HwFaultCode_enum"
  VMIN_Dir_PlatformFaultMask_u32/1 -> Bus Creator2/12  "VMIN_Dir_PlatformFaultMask_u32"
  VMIN_Dir_PlatformWarningMask_u32/1 -> Bus Creator2/13  "VMIN_Dir_PlatformWarningMask_u32"
  PlatformTorqueLimit/1 -> Bus Creator2/14  "VMIN_Dir_PlatformTorqueLimitFactor_NULL"

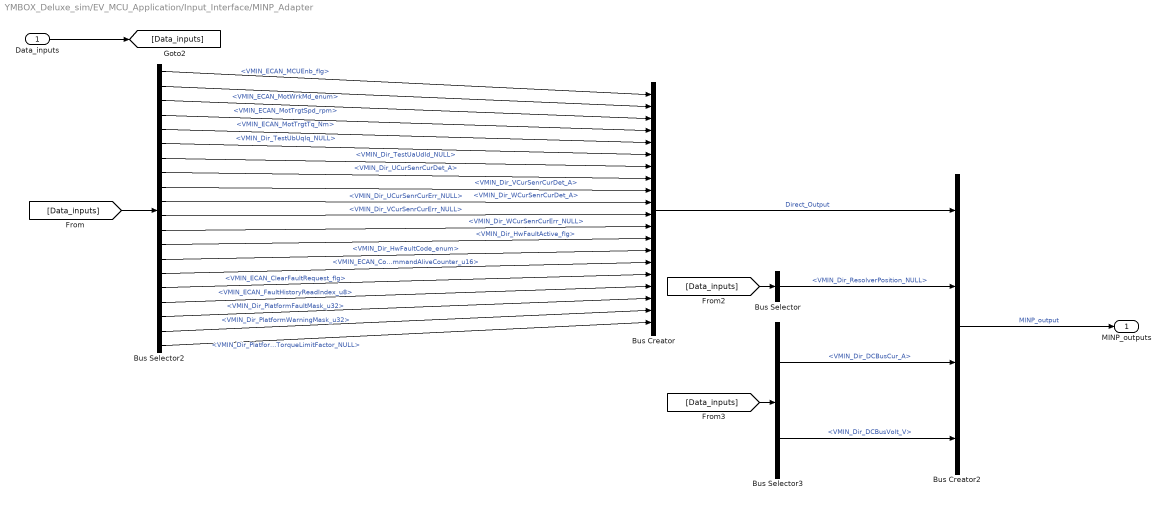
== system YMBOX_Deluxe_sim/EV_MCU_Application/Input_Interface/MINP_Adapter ==
  Data_inputs : Inport
  Bus Creator : BusCreator  Inputs=20  OutDataTypeStr=Bus: Direct_Output  NonVirtualBus=on
      settings: InheritFromInputs=off
  Bus Creator2 : BusCreator  Inputs=4  OutDataTypeStr=Bus: MINP_output  NonVirtualBus=on
      settings: InheritFromInputs=off
  Bus Selector : BusSelector  OutputSignals=signal1.MCU_Direct_Bottom_Input.VMIN_Dir_ResolverPosition_NULL
  Bus Selector2 : BusSelector  OutputSignals=signal2.EVCAN_Input.VMIN_ECAN_MCUEnb_flg,signal2.EVCAN_Input.VMIN_ECAN_MotWrkMd_enum,signal2.EVCAN_Input.VMIN_ECAN_MotTrgtSpd_rpm,signal2.EVCAN_Input.VMIN_ECAN_MotTrgtTq_Nm,signal1.MCU_Direct_Bottom_Input.VMIN_Dir_TestUbUqIq_NULL,signal1.MCU_Direct_Bottom_Input.VMIN_Dir_TestUaUdId_NULL,signal1.MCU_Direct_Bottom_Input.VMIN_Dir_UCurSenrCurDet_A,signal1.MCU_Direct_Bottom_Input.VMIN_Dir_VCurSenrCurDet_A,signal1.MCU_Direct_Bottom_Input.VMIN_Dir_WCurSenrCurDet_A,signal1.MCU_Direct_Bottom_Input.VMIN_Dir_UCurSenrCurErr_NULL,signal1.MCU_Direct_Bottom_Input.VMIN_Dir_VCurSenrCurErr_NULL,signal1.MCU_Direct_Bottom_Input.VMIN_Dir_WCurSenrCurErr_NULL,signal1.MCU_Direct_Bottom_Input.VMIN_Dir_HwFaultActive_flg,signal1.MCU_Direct_Bottom_Input.VMIN_Dir_HwFaultCode_enum,signal2.EVCAN_Input.VMIN_ECAN_CommandAliveCounter_u16,signal2.EVCAN_Input.VMIN_ECAN_ClearFaultRequest_flg,signal2.EVCAN_Input.VMIN_ECAN_FaultHistoryReadIndex_u8,signal1.MCU_Direct_Bottom_Input.VMIN_Dir_PlatformFaultMask_u32,signal1.MCU_Direct_Bottom_Input.VMIN_Dir_PlatformWarningMask_u32,signal1.MCU_Direct_Bottom_Input.VMIN_Dir_PlatformTorqueLimitFactor_NULL
  Bus Selector3 : BusSelector  OutputSignals=signal1.MCU_Direct_Adc_Input.VMIN_Dir_DCBusCur_A,signal1.MCU_Direct_Adc_Input.VMIN_Dir_DCBusVolt_V
  MINP_outputs : Outport  OutDataTypeStr=Bus: MINP_output
  wires:
  Data_inputs/1 -> [Data_inputs]
  [Data_inputs] -> Bus Selector2/1
  Bus Selector2/1 -> Bus Creator/1  "<VMIN_ECAN_MCUEnb_flg>"
  Bus Selector2/2 -> Bus Creator/2  "<VMIN_ECAN_MotWrkMd_enum>"
  Bus Selector2/3 -> Bus Creator/3  "<VMIN_ECAN_MotTrgtSpd_rpm>"
  Bus Selector2/5 -> Bus Creator/5  "<VMIN_Dir_TestUbUqIq_NULL>"
  Bus Selector2/6 -> Bus Creator/6  "<VMIN_Dir_TestUaUdId_NULL>"
  Bus Selector2/7 -> Bus Creator/7  "<VMIN_Dir_UCurSenrCurDet_A>"
  Bus Selector2/8 -> Bus Creator/8  "<VMIN_Dir_VCurSenrCurDet_A>"
  Bus Selector2/9 -> Bus Creator/9  "<VMIN_Dir_WCurSenrCurDet_A>"
  [Data_inputs] -> Bus Selector3/1
  Bus Selector2/4 -> Bus Creator/4  "<VMIN_ECAN_MotTrgtTq_Nm>"
  Bus Creator/1 -> Bus Creator2/1  "Direct_Output"
  Bus Creator2/1 -> MINP_outputs/1  "MINP_output"
  [Data_inputs] -> Bus Selector/1
  Bus Selector2/10 -> Bus Creator/10  "<VMIN_Dir_UCurSenrCurErr_NULL>"
  Bus Selector2/11 -> Bus Creator/11  "<VMIN_Dir_VCurSenrCurErr_NULL>"
  Bus Selector2/12 -> Bus Creator/12  "<VMIN_Dir_WCurSenrCurErr_NULL>"
  Bus Selector2/13 -> Bus Creator/13  "<VMIN_Dir_HwFaultActive_flg>"
  Bus Selector2/14 -> Bus Creator/14  "<VMIN_Dir_HwFaultCode_enum>"
  Bus Selector2/15 -> Bus Creator/15  "<VMIN_ECAN_CommandAliveCounter_u16>"
  Bus Selector2/16 -> Bus Creator/16  "<VMIN_ECAN_ClearFaultRequest_flg>"
  Bus Selector2/17 -> Bus Creator/17  "<VMIN_ECAN_FaultHistoryReadIndex_u8>"
  Bus Selector2/18 -> Bus Creator/18  "<VMIN_Dir_PlatformFaultMask_u32>"
  Bus Selector2/19 -> Bus Creator/19  "<VMIN_Dir_PlatformWarningMask_u32>"
  Bus Selector2/20 -> Bus Creator/20  "<VMIN_Dir_PlatformTorqueLimitFactor_NULL>"
  Bus Selector/1 -> Bus Creator2/2  "<VMIN_Dir_ResolverPosition_NULL>"
  Bus Selector3/1 -> Bus Creator2/3  "<VMIN_Dir_DCBusCur_A>"
  Bus Selector3/2 -> Bus Creator2/4  "<VMIN_Dir_DCBusVolt_V>"

== stateflow chart YMBOX_Deluxe_sim/EV_MCU_Application/Application_Scheduler/Application_Scheduler_Chart ==
  settings: updateMethod=DISCRETE  sampleTime=Cf_CONTROL_TASK_TIME_S
  (default) -> (junction 113)
  (junction 113) -> (junction 114) : {
      |   Data_Inputs_Call;
      |   MCU_App_Strategy_Call;
      | }
  events: MCU_App_Strategy_Call output FUNCTION_CALL_EVENT; Data_Inputs_Call output FUNCTION_CALL_EVENT
